simulink model "shc_two_masses"  (R2023a)
settings: Solver=FixedStepDiscrete  StartTime=0.0  StopTime=200  FixedStep=0.01  RelTol=1e-3
undefined symbols (not defined in the file or in its folder): DiscIntNeverNeededParam
libraries: SHCLib x1
settings Model: Creator=hwx20  LastModifiedBy=hwx20

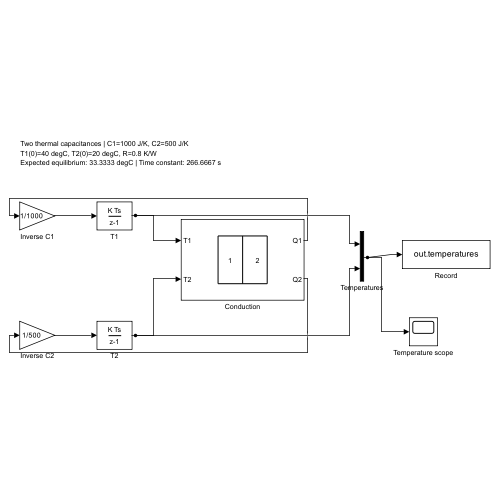
[thumbnail: Simulink's stored preview of the top-level diagram]
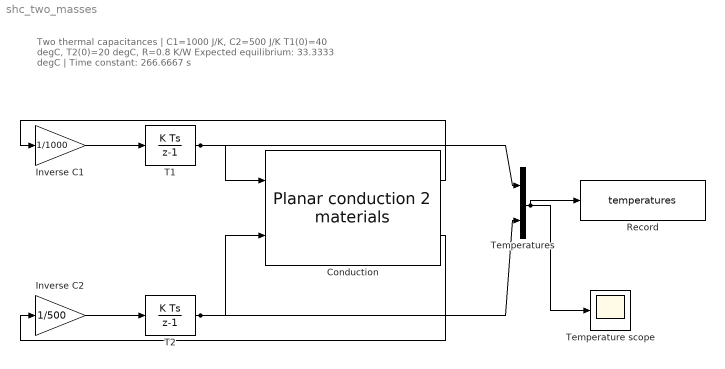
== system shc_two_masses ==
  note: Two thermal capacitances | C1=1000 J/K, C2=500 J/K
      | T1(0)=40 degC, T2(0)=20 degC, R=0.8 K/W
      | Expected equilibrium: 33.3333 degC | Time constant: 266.6667 s
  Conduction : SHCLib/Planar conduction 2 materials  lambda1=1  distance1=0.005  lambda2=2  distance2=0.002  area=0.01  ctr=0.2
      settings: SourceProductName=Heat Conduction
  Inverse C1 : Gain  Gain=1/1000
  Inverse C2 : Gain  Gain=1/500
  Record : ToWorkspace  VariableName=temperatures  SaveFormat=Structure With Time  SampleTime=-1
  T1 : DiscreteIntegrator  InitialCondition=40  SampleTime=0.01  ICPrevOutput=DiscIntNeverNeededParam  ICPrevScaledInput=DiscIntNeverNeededParam
  T2 : DiscreteIntegrator  InitialCondition=20  SampleTime=0.01  ICPrevOutput=DiscIntNeverNeededParam  ICPrevScaledInput=DiscIntNeverNeededParam
  Temperature scope : Scope
  Temperatures : Mux  Inputs=2
  wires:
  T1/1 -> Conduction/1, Temperatures/1
  T2/1 -> Conduction/2, Temperatures/2
  Conduction/1 -> Inverse C1/1
  Conduction/2 -> Inverse C2/1
  Inverse C1/1 -> T1/1
  Inverse C2/1 -> T2/1
  Temperatures/1 -> Record/1, Temperature scope/1
